simulink model "TB23_R2_SALS_Link"  (R2025a)
settings: Solver=FixedStepDiscrete  StartTime=0  StopTime=TB.t_end  FixedStep=TB.dt  RelTol=1e-3
InitFcn:
  | % 모델과 같은 폴더의 초기화 스크립트를 실행해 P(설계 파라미터)와 TB(시험 조건)를 만든다.
  | run(fullfile(fileparts(get_param(bdroot, 'FileName')), 'TB23_init.m'));
values from neighbouring files (symbols this model uses):
  TB = struct()    [TB23_init.m]    (also in run_TB23.m = evalin('base', 'TB'))
libraries: fl_lib x71, nesl_utility x31
(part 2 of 3)

== system TB23_R2_SALS_Link/StageB_Regulator/DAB_Primary/P3_leg2_high ==
  note: 스위치 셀: 이상 스위치(R_on, G_off) + 역병렬 바디 다이오드(Vf, R_d) + 출력용량 C_oss
      | 게이트: 전역 태그 "gD_P3" (> 0.5 이면 도통)
  C_oss : fl_lib/Electrical/Electrical Elements/Capacitor  c=Coss F  r=1e-6 Ohm  g=0 1/Ohm  i_specify=off  i_priority=None  i=0 A  i_nominal_specify=off  i_nominal_value=1  i_nominal_unit=A  v_specify=off  v_priority=None  v=0 V  v_nominal_specify=off  v_nominal_value=1  v_nominal_unit=V  vc_specify=off  vc_priority=High  vc=0 V  vc_nominal_specify=off  vc_nominal_value=1  vc_nominal_unit=V
  D_body : fl_lib/Electrical/Electrical Elements/Diode  Vf=Vf V  Ron=Rd Ohm  Goff=Goffd 1/Ohm  i_specify=off  i_priority=None  i=0 A  i_nominal_specify=off  i_nominal_value=1  i_nominal_unit=A  v_specify=off  v_priority=None  v=0 V  v_nominal_specify=off  v_nominal_value=1  v_nominal_unit=V
  Gate_PS : nesl_utility/Simulink-PS Converter  PhysicalDomain=network_engine_domain  SubClassName=ps_input  LeftPortType=input  RightPortType=output  PseudoPeriodic=off  Frequencies=[]  NoiseDistribution=none  NoiseParameters=[]  Unit=1  AffineConversion=off  FilteringAndDerivatives=zero  SimscapeFilterOrder=1  InputFilterTimeConstant=0.001  UdotUserProvided=0
  SW : fl_lib/Electrical/Electrical Elements/Switch  R_closed=Ron Ohm  G_open=Goff 1/Ohm  Threshold=0.5  i_specify=off  i_priority=None  i=0 A  i_nominal_specify=off  i_nominal_value=1  i_nominal_unit=A  v_specify=off  v_priority=None  v=0 V  v_nominal_specify=off  v_nominal_value=1  v_nominal_unit=V
  D : PMIOPort  Side=Left
  S : PMIOPort  Port=2  Side=Right
  wires:
  [gD_P3] -> Gate_PS/1
  connections:
  Gate_PS/RConn1 -- SW/RConn1
  SW/LConn1 -- D/RConn1 -- D_body/RConn1 -- C_oss/LConn1
  SW/RConn2 -- D_body/LConn1 -- S/RConn1 -- C_oss/RConn1

== system TB23_R2_SALS_Link/StageB_Regulator/DAB_Primary/P4_leg2_low ==
  note: 스위치 셀: 이상 스위치(R_on, G_off) + 역병렬 바디 다이오드(Vf, R_d) + 출력용량 C_oss
      | 게이트: 전역 태그 "gD_P4" (> 0.5 이면 도통)
  C_oss : fl_lib/Electrical/Electrical Elements/Capacitor  c=Coss F  r=1e-6 Ohm  g=0 1/Ohm  i_specify=off  i_priority=None  i=0 A  i_nominal_specify=off  i_nominal_value=1  i_nominal_unit=A  v_specify=off  v_priority=None  v=0 V  v_nominal_specify=off  v_nominal_value=1  v_nominal_unit=V  vc_specify=off  vc_priority=High  vc=0 V  vc_nominal_specify=off  vc_nominal_value=1  vc_nominal_unit=V
  D_body : fl_lib/Electrical/Electrical Elements/Diode  Vf=Vf V  Ron=Rd Ohm  Goff=Goffd 1/Ohm  i_specify=off  i_priority=None  i=0 A  i_nominal_specify=off  i_nominal_value=1  i_nominal_unit=A  v_specify=off  v_priority=None  v=0 V  v_nominal_specify=off  v_nominal_value=1  v_nominal_unit=V
  Gate_PS : nesl_utility/Simulink-PS Converter  PhysicalDomain=network_engine_domain  SubClassName=ps_input  LeftPortType=input  RightPortType=output  PseudoPeriodic=off  Frequencies=[]  NoiseDistribution=none  NoiseParameters=[]  Unit=1  AffineConversion=off  FilteringAndDerivatives=zero  SimscapeFilterOrder=1  InputFilterTimeConstant=0.001  UdotUserProvided=0
  SW : fl_lib/Electrical/Electrical Elements/Switch  R_closed=Ron Ohm  G_open=Goff 1/Ohm  Threshold=0.5  i_specify=off  i_priority=None  i=0 A  i_nominal_specify=off  i_nominal_value=1  i_nominal_unit=A  v_specify=off  v_priority=None  v=0 V  v_nominal_specify=off  v_nominal_value=1  v_nominal_unit=V
  D : PMIOPort  Side=Left
  S : PMIOPort  Port=2  Side=Right
  wires:
  [gD_P4] -> Gate_PS/1
  connections:
  Gate_PS/RConn1 -- SW/RConn1
  SW/LConn1 -- D/RConn1 -- D_body/RConn1 -- C_oss/LConn1
  SW/RConn2 -- D_body/LConn1 -- S/RConn1 -- C_oss/RConn1

== system TB23_R2_SALS_Link/StageB_Regulator/DAB_Secondary/S1_leg1_high ==
  note: 스위치 셀: 이상 스위치(R_on, G_off) + 역병렬 바디 다이오드(Vf, R_d) + 출력용량 C_oss
      | 게이트: 전역 태그 "gD_S1" (> 0.5 이면 도통)
  C_oss : fl_lib/Electrical/Electrical Elements/Capacitor  c=Coss F  r=1e-6 Ohm  g=0 1/Ohm  i_specify=off  i_priority=None  i=0 A  i_nominal_specify=off  i_nominal_value=1  i_nominal_unit=A  v_specify=off  v_priority=None  v=0 V  v_nominal_specify=off  v_nominal_value=1  v_nominal_unit=V  vc_specify=off  vc_priority=High  vc=0 V  vc_nominal_specify=off  vc_nominal_value=1  vc_nominal_unit=V
  D_body : fl_lib/Electrical/Electrical Elements/Diode  Vf=Vf V  Ron=Rd Ohm  Goff=Goffd 1/Ohm  i_specify=off  i_priority=None  i=0 A  i_nominal_specify=off  i_nominal_value=1  i_nominal_unit=A  v_specify=off  v_priority=None  v=0 V  v_nominal_specify=off  v_nominal_value=1  v_nominal_unit=V
  Gate_PS : nesl_utility/Simulink-PS Converter  PhysicalDomain=network_engine_domain  SubClassName=ps_input  LeftPortType=input  RightPortType=output  PseudoPeriodic=off  Frequencies=[]  NoiseDistribution=none  NoiseParameters=[]  Unit=1  AffineConversion=off  FilteringAndDerivatives=zero  SimscapeFilterOrder=1  InputFilterTimeConstant=0.001  UdotUserProvided=0
  SW : fl_lib/Electrical/Electrical Elements/Switch  R_closed=Ron Ohm  G_open=Goff 1/Ohm  Threshold=0.5  i_specify=off  i_priority=None  i=0 A  i_nominal_specify=off  i_nominal_value=1  i_nominal_unit=A  v_specify=off  v_priority=None  v=0 V  v_nominal_specify=off  v_nominal_value=1  v_nominal_unit=V
  D : PMIOPort  Side=Left
  S : PMIOPort  Port=2  Side=Right
  wires:
  [gD_S1] -> Gate_PS/1
  connections:
  Gate_PS/RConn1 -- SW/RConn1
  SW/LConn1 -- D/RConn1 -- D_body/RConn1 -- C_oss/LConn1
  SW/RConn2 -- D_body/LConn1 -- S/RConn1 -- C_oss/RConn1

== system TB23_R2_SALS_Link/StageB_Regulator/DAB_Secondary/S2_leg1_low ==
  note: 스위치 셀: 이상 스위치(R_on, G_off) + 역병렬 바디 다이오드(Vf, R_d) + 출력용량 C_oss
      | 게이트: 전역 태그 "gD_S2" (> 0.5 이면 도통)
  C_oss : fl_lib/Electrical/Electrical Elements/Capacitor  c=Coss F  r=1e-6 Ohm  g=0 1/Ohm  i_specify=off  i_priority=None  i=0 A  i_nominal_specify=off  i_nominal_value=1  i_nominal_unit=A  v_specify=off  v_priority=None  v=0 V  v_nominal_specify=off  v_nominal_value=1  v_nominal_unit=V  vc_specify=off  vc_priority=High  vc=0 V  vc_nominal_specify=off  vc_nominal_value=1  vc_nominal_unit=V
  D_body : fl_lib/Electrical/Electrical Elements/Diode  Vf=Vf V  Ron=Rd Ohm  Goff=Goffd 1/Ohm  i_specify=off  i_priority=None  i=0 A  i_nominal_specify=off  i_nominal_value=1  i_nominal_unit=A  v_specify=off  v_priority=None  v=0 V  v_nominal_specify=off  v_nominal_value=1  v_nominal_unit=V
  Gate_PS : nesl_utility/Simulink-PS Converter  PhysicalDomain=network_engine_domain  SubClassName=ps_input  LeftPortType=input  RightPortType=output  PseudoPeriodic=off  Frequencies=[]  NoiseDistribution=none  NoiseParameters=[]  Unit=1  AffineConversion=off  FilteringAndDerivatives=zero  SimscapeFilterOrder=1  InputFilterTimeConstant=0.001  UdotUserProvided=0
  SW : fl_lib/Electrical/Electrical Elements/Switch  R_closed=Ron Ohm  G_open=Goff 1/Ohm  Threshold=0.5  i_specify=off  i_priority=None  i=0 A  i_nominal_specify=off  i_nominal_value=1  i_nominal_unit=A  v_specify=off  v_priority=None  v=0 V  v_nominal_specify=off  v_nominal_value=1  v_nominal_unit=V
  D : PMIOPort  Side=Left
  S : PMIOPort  Port=2  Side=Right
  wires:
  [gD_S2] -> Gate_PS/1
  connections:
  Gate_PS/RConn1 -- SW/RConn1
  SW/LConn1 -- D/RConn1 -- D_body/RConn1 -- C_oss/LConn1
  SW/RConn2 -- D_body/LConn1 -- S/RConn1 -- C_oss/RConn1

== system TB23_R2_SALS_Link/StageB_Regulator/DAB_Secondary/S3_leg2_high ==
  note: 스위치 셀: 이상 스위치(R_on, G_off) + 역병렬 바디 다이오드(Vf, R_d) + 출력용량 C_oss
      | 게이트: 전역 태그 "gD_S3" (> 0.5 이면 도통)
  C_oss : fl_lib/Electrical/Electrical Elements/Capacitor  c=Coss F  r=1e-6 Ohm  g=0 1/Ohm  i_specify=off  i_priority=None  i=0 A  i_nominal_specify=off  i_nominal_value=1  i_nominal_unit=A  v_specify=off  v_priority=None  v=0 V  v_nominal_specify=off  v_nominal_value=1  v_nominal_unit=V  vc_specify=off  vc_priority=High  vc=0 V  vc_nominal_specify=off  vc_nominal_value=1  vc_nominal_unit=V
  D_body : fl_lib/Electrical/Electrical Elements/Diode  Vf=Vf V  Ron=Rd Ohm  Goff=Goffd 1/Ohm  i_specify=off  i_priority=None  i=0 A  i_nominal_specify=off  i_nominal_value=1  i_nominal_unit=A  v_specify=off  v_priority=None  v=0 V  v_nominal_specify=off  v_nominal_value=1  v_nominal_unit=V
  Gate_PS : nesl_utility/Simulink-PS Converter  PhysicalDomain=network_engine_domain  SubClassName=ps_input  LeftPortType=input  RightPortType=output  PseudoPeriodic=off  Frequencies=[]  NoiseDistribution=none  NoiseParameters=[]  Unit=1  AffineConversion=off  FilteringAndDerivatives=zero  SimscapeFilterOrder=1  InputFilterTimeConstant=0.001  UdotUserProvided=0
  SW : fl_lib/Electrical/Electrical Elements/Switch  R_closed=Ron Ohm  G_open=Goff 1/Ohm  Threshold=0.5  i_specify=off  i_priority=None  i=0 A  i_nominal_specify=off  i_nominal_value=1  i_nominal_unit=A  v_specify=off  v_priority=None  v=0 V  v_nominal_specify=off  v_nominal_value=1  v_nominal_unit=V
  D : PMIOPort  Side=Left
  S : PMIOPort  Port=2  Side=Right
  wires:
  [gD_S3] -> Gate_PS/1
  connections:
  Gate_PS/RConn1 -- SW/RConn1
  SW/LConn1 -- D/RConn1 -- D_body/RConn1 -- C_oss/LConn1
  SW/RConn2 -- D_body/LConn1 -- S/RConn1 -- C_oss/RConn1

== system TB23_R2_SALS_Link/StageB_Regulator/DAB_Secondary/S4_leg2_low ==
  note: 스위치 셀: 이상 스위치(R_on, G_off) + 역병렬 바디 다이오드(Vf, R_d) + 출력용량 C_oss
      | 게이트: 전역 태그 "gD_S4" (> 0.5 이면 도통)
  C_oss : fl_lib/Electrical/Electrical Elements/Capacitor  c=Coss F  r=1e-6 Ohm  g=0 1/Ohm  i_specify=off  i_priority=None  i=0 A  i_nominal_specify=off  i_nominal_value=1  i_nominal_unit=A  v_specify=off  v_priority=None  v=0 V  v_nominal_specify=off  v_nominal_value=1  v_nominal_unit=V  vc_specify=off  vc_priority=High  vc=0 V  vc_nominal_specify=off  vc_nominal_value=1  vc_nominal_unit=V
  D_body : fl_lib/Electrical/Electrical Elements/Diode  Vf=Vf V  Ron=Rd Ohm  Goff=Goffd 1/Ohm  i_specify=off  i_priority=None  i=0 A  i_nominal_specify=off  i_nominal_value=1  i_nominal_unit=A  v_specify=off  v_priority=None  v=0 V  v_nominal_specify=off  v_nominal_value=1  v_nominal_unit=V
  Gate_PS : nesl_utility/Simulink-PS Converter  PhysicalDomain=network_engine_domain  SubClassName=ps_input  LeftPortType=input  RightPortType=output  PseudoPeriodic=off  Frequencies=[]  NoiseDistribution=none  NoiseParameters=[]  Unit=1  AffineConversion=off  FilteringAndDerivatives=zero  SimscapeFilterOrder=1  InputFilterTimeConstant=0.001  UdotUserProvided=0
  SW : fl_lib/Electrical/Electrical Elements/Switch  R_closed=Ron Ohm  G_open=Goff 1/Ohm  Threshold=0.5  i_specify=off  i_priority=None  i=0 A  i_nominal_specify=off  i_nominal_value=1  i_nominal_unit=A  v_specify=off  v_priority=None  v=0 V  v_nominal_specify=off  v_nominal_value=1  v_nominal_unit=V
  D : PMIOPort  Side=Left
  S : PMIOPort  Port=2  Side=Right
  wires:
  [gD_S4] -> Gate_PS/1
  connections:
  Gate_PS/RConn1 -- SW/RConn1
  SW/LConn1 -- D/RConn1 -- D_body/RConn1 -- C_oss/LConn1
  SW/RConn2 -- D_body/LConn1 -- S/RConn1 -- C_oss/RConn1

== system TB23_R2_SALS_Link/StageB_Regulator/HBridge/QA_high ==
  note: 스위치 셀: 이상 스위치(R_on, G_off) + 역병렬 바디 다이오드(Vf, R_d) + 출력용량 C_oss
      | 게이트: 전역 태그 "gB_AH" (> 0.5 이면 도통)
  C_oss : fl_lib/Electrical/Electrical Elements/Capacitor  c=Coss F  r=1e-6 Ohm  g=0 1/Ohm  i_specify=off  i_priority=None  i=0 A  i_nominal_specify=off  i_nominal_value=1  i_nominal_unit=A  v_specify=off  v_priority=None  v=0 V  v_nominal_specify=off  v_nominal_value=1  v_nominal_unit=V  vc_specify=off  vc_priority=High  vc=0 V  vc_nominal_specify=off  vc_nominal_value=1  vc_nominal_unit=V
  D_body : fl_lib/Electrical/Electrical Elements/Diode  Vf=Vf V  Ron=Rd Ohm  Goff=Goffd 1/Ohm  i_specify=off  i_priority=None  i=0 A  i_nominal_specify=off  i_nominal_value=1  i_nominal_unit=A  v_specify=off  v_priority=None  v=0 V  v_nominal_specify=off  v_nominal_value=1  v_nominal_unit=V
  Gate_PS : nesl_utility/Simulink-PS Converter  PhysicalDomain=network_engine_domain  SubClassName=ps_input  LeftPortType=input  RightPortType=output  PseudoPeriodic=off  Frequencies=[]  NoiseDistribution=none  NoiseParameters=[]  Unit=1  AffineConversion=off  FilteringAndDerivatives=zero  SimscapeFilterOrder=1  InputFilterTimeConstant=0.001  UdotUserProvided=0
  SW : fl_lib/Electrical/Electrical Elements/Switch  R_closed=Ron Ohm  G_open=Goff 1/Ohm  Threshold=0.5  i_specify=off  i_priority=None  i=0 A  i_nominal_specify=off  i_nominal_value=1  i_nominal_unit=A  v_specify=off  v_priority=None  v=0 V  v_nominal_specify=off  v_nominal_value=1  v_nominal_unit=V
  D : PMIOPort  Side=Left
  S : PMIOPort  Port=2  Side=Right
  wires:
  [gB_AH] -> Gate_PS/1
  connections:
  Gate_PS/RConn1 -- SW/RConn1
  SW/LConn1 -- D/RConn1 -- D_body/RConn1 -- C_oss/LConn1
  SW/RConn2 -- D_body/LConn1 -- S/RConn1 -- C_oss/RConn1

== system TB23_R2_SALS_Link/StageB_Regulator/HBridge/QA_low ==
  note: 스위치 셀: 이상 스위치(R_on, G_off) + 역병렬 바디 다이오드(Vf, R_d) + 출력용량 C_oss
      | 게이트: 전역 태그 "gB_AL" (> 0.5 이면 도통)
  C_oss : fl_lib/Electrical/Electrical Elements/Capacitor  c=Coss F  r=1e-6 Ohm  g=0 1/Ohm  i_specify=off  i_priority=None  i=0 A  i_nominal_specify=off  i_nominal_value=1  i_nominal_unit=A  v_specify=off  v_priority=None  v=0 V  v_nominal_specify=off  v_nominal_value=1  v_nominal_unit=V  vc_specify=off  vc_priority=High  vc=0 V  vc_nominal_specify=off  vc_nominal_value=1  vc_nominal_unit=V
  D_body : fl_lib/Electrical/Electrical Elements/Diode  Vf=Vf V  Ron=Rd Ohm  Goff=Goffd 1/Ohm  i_specify=off  i_priority=None  i=0 A  i_nominal_specify=off  i_nominal_value=1  i_nominal_unit=A  v_specify=off  v_priority=None  v=0 V  v_nominal_specify=off  v_nominal_value=1  v_nominal_unit=V
  Gate_PS : nesl_utility/Simulink-PS Converter  PhysicalDomain=network_engine_domain  SubClassName=ps_input  LeftPortType=input  RightPortType=output  PseudoPeriodic=off  Frequencies=[]  NoiseDistribution=none  NoiseParameters=[]  Unit=1  AffineConversion=off  FilteringAndDerivatives=zero  SimscapeFilterOrder=1  InputFilterTimeConstant=0.001  UdotUserProvided=0
  SW : fl_lib/Electrical/Electrical Elements/Switch  R_closed=Ron Ohm  G_open=Goff 1/Ohm  Threshold=0.5  i_specify=off  i_priority=None  i=0 A  i_nominal_specify=off  i_nominal_value=1  i_nominal_unit=A  v_specify=off  v_priority=None  v=0 V  v_nominal_specify=off  v_nominal_value=1  v_nominal_unit=V
  D : PMIOPort  Side=Left
  S : PMIOPort  Port=2  Side=Right
  wires:
  [gB_AL] -> Gate_PS/1
  connections:
  Gate_PS/RConn1 -- SW/RConn1
  SW/LConn1 -- D/RConn1 -- D_body/RConn1 -- C_oss/LConn1
  SW/RConn2 -- D_body/LConn1 -- S/RConn1 -- C_oss/RConn1

== system TB23_R2_SALS_Link/StageB_Regulator/HBridge/QB_high ==
  note: 스위치 셀: 이상 스위치(R_on, G_off) + 역병렬 바디 다이오드(Vf, R_d) + 출력용량 C_oss
      | 게이트: 전역 태그 "gB_BH" (> 0.5 이면 도통)
  C_oss : fl_lib/Electrical/Electrical Elements/Capacitor  c=Coss F  r=1e-6 Ohm  g=0 1/Ohm  i_specify=off  i_priority=None  i=0 A  i_nominal_specify=off  i_nominal_value=1  i_nominal_unit=A  v_specify=off  v_priority=None  v=0 V  v_nominal_specify=off  v_nominal_value=1  v_nominal_unit=V  vc_specify=off  vc_priority=High  vc=0 V  vc_nominal_specify=off  vc_nominal_value=1  vc_nominal_unit=V
  D_body : fl_lib/Electrical/Electrical Elements/Diode  Vf=Vf V  Ron=Rd Ohm  Goff=Goffd 1/Ohm  i_specify=off  i_priority=None  i=0 A  i_nominal_specify=off  i_nominal_value=1  i_nominal_unit=A  v_specify=off  v_priority=None  v=0 V  v_nominal_specify=off  v_nominal_value=1  v_nominal_unit=V
  Gate_PS : nesl_utility/Simulink-PS Converter  PhysicalDomain=network_engine_domain  SubClassName=ps_input  LeftPortType=input  RightPortType=output  PseudoPeriodic=off  Frequencies=[]  NoiseDistribution=none  NoiseParameters=[]  Unit=1  AffineConversion=off  FilteringAndDerivatives=zero  SimscapeFilterOrder=1  InputFilterTimeConstant=0.001  UdotUserProvided=0
  SW : fl_lib/Electrical/Electrical Elements/Switch  R_closed=Ron Ohm  G_open=Goff 1/Ohm  Threshold=0.5  i_specify=off  i_priority=None  i=0 A  i_nominal_specify=off  i_nominal_value=1  i_nominal_unit=A  v_specify=off  v_priority=None  v=0 V  v_nominal_specify=off  v_nominal_value=1  v_nominal_unit=V
  D : PMIOPort  Side=Left
  S : PMIOPort  Port=2  Side=Right
  wires:
  [gB_BH] -> Gate_PS/1
  connections:
  Gate_PS/RConn1 -- SW/RConn1
  SW/LConn1 -- D/RConn1 -- D_body/RConn1 -- C_oss/LConn1
  SW/RConn2 -- D_body/LConn1 -- S/RConn1 -- C_oss/RConn1

== system TB23_R2_SALS_Link/StageB_Regulator/HBridge/QB_low ==
  note: 스위치 셀: 이상 스위치(R_on, G_off) + 역병렬 바디 다이오드(Vf, R_d) + 출력용량 C_oss
      | 게이트: 전역 태그 "gB_BL" (> 0.5 이면 도통)
  C_oss : fl_lib/Electrical/Electrical Elements/Capacitor  c=Coss F  r=1e-6 Ohm  g=0 1/Ohm  i_specify=off  i_priority=None  i=0 A  i_nominal_specify=off  i_nominal_value=1  i_nominal_unit=A  v_specify=off  v_priority=None  v=0 V  v_nominal_specify=off  v_nominal_value=1  v_nominal_unit=V  vc_specify=off  vc_priority=High  vc=0 V  vc_nominal_specify=off  vc_nominal_value=1  vc_nominal_unit=V
  D_body : fl_lib/Electrical/Electrical Elements/Diode  Vf=Vf V  Ron=Rd Ohm  Goff=Goffd 1/Ohm  i_specify=off  i_priority=None  i=0 A  i_nominal_specify=off  i_nominal_value=1  i_nominal_unit=A  v_specify=off  v_priority=None  v=0 V  v_nominal_specify=off  v_nominal_value=1  v_nominal_unit=V
  Gate_PS : nesl_utility/Simulink-PS Converter  PhysicalDomain=network_engine_domain  SubClassName=ps_input  LeftPortType=input  RightPortType=output  PseudoPeriodic=off  Frequencies=[]  NoiseDistribution=none  NoiseParameters=[]  Unit=1  AffineConversion=off  FilteringAndDerivatives=zero  SimscapeFilterOrder=1  InputFilterTimeConstant=0.001  UdotUserProvided=0
  SW : fl_lib/Electrical/Electrical Elements/Switch  R_closed=Ron Ohm  G_open=Goff 1/Ohm  Threshold=0.5  i_specify=off  i_priority=None  i=0 A  i_nominal_specify=off  i_nominal_value=1  i_nominal_unit=A  v_specify=off  v_priority=None  v=0 V  v_nominal_specify=off  v_nominal_value=1  v_nominal_unit=V
  D : PMIOPort  Side=Left
  S : PMIOPort  Port=2  Side=Right
  wires:
  [gB_BL] -> Gate_PS/1
  connections:
  Gate_PS/RConn1 -- SW/RConn1
  SW/LConn1 -- D/RConn1 -- D_body/RConn1 -- C_oss/LConn1
  SW/RConn2 -- D_body/LConn1 -- S/RConn1 -- C_oss/RConn1

== matlab function TB23_R2_SALS_Link/Load_CPL/SALS_Loads ==
  data: t input; i_load output; vb input; code input; prm input; p_load output
function [i_load, p_load] = prism_sals_loads(t, vb, code, prm)
%#codegen
%PRISM_SALS_LOADS  400 V 부하의 등급별 계약 응답(SALS 메시지 지연·손실·워치독 포함). TB23부터.
%
%   검증 코드 sals_loads.SalsLoads(E29)와 같은 해석식이다. 보호 상태기계(ctrl/prism_r2_supervisor.m, SALS 모드)가
%   s(10)에 비트로 명령을 낸다: 1 접촉기 열림(400 V급 부하 분리), 2 SALS 감발, 4 SALS 되돌림, 8 Stage C 회생 차단,
%   16 Stage A 정지(이 블록은 쓰지 않음). 비트가 처음 켜진 시각을 명령 시각으로 잡는다.
%     M0  Stage C sc(회생 차단이면 t_sc 뒤 하한 0으로 sc_slew 변화율), V2L v2l(계단, SALS로 줄이지 않음)
%     M1  컴프레서 comp, D  PTC ptc·배터리 히터 bh:
%         감발 도착 = 명령 + 재송신 주기 × (앞의 손실 수) + 지연. 손실 수 −1이면 모두 손실(도착 없음).
%         D는 워치독으로 명령 + wd에 0으로 간다(마지막 유효 수신 ≤ 명령 시각). 도착 뒤 감소 변화율 dn으로 0까지.
%         되돌림 도착 뒤 증가 변화율 up으로 요청값까지(되돌림이 감발보다 먼저 도착하면 감발은 버려진다).
%     접촉기 열림이면 Stage C만 남는다. 버스가 v_cut 아래면 모든 부하가 끊긴다(검증 코드 E17의 저전압 차단).
%
%   입력  t 시각 [s], vb 버스전압(한 간격 지연·시작 보호), code s(10) 비트 명령,
%         prm [sc v2l comp ptc bh | d_comp d_ptc d_bh | k_comp k_ptc k_bh | kr_comp kr_ptc kr_bh |
%              period wd up dn t_sc sc_slew v_min v_cut]  (22개, 시간 [s]·변화율 [W/s]는 시간 축소를 이미 넣은 값)
%   출력  i_load = p_load / max(vb, v_min) [A], p_load [W]

persistent t_cut t_rest t_blk acut arest
if isempty(t_cut)
    t_cut = -1; t_rest = -1; t_blk = -1; acut = inf(3, 1); arest = inf(3, 1);
end
mix = prm(1:5); dl = prm(6:8); kc = prm(9:11); kr = prm(12:14);
period = prm(15); wd = prm(16); up = prm(17); dn = prm(18); t_sc = prm(19); sc_slew = prm(20); vmin = prm(21); vcut = prm(22);
c = round(code);
open_c = mod(c, 2) >= 1; cut = mod(floor(c/2), 2) >= 1; rest = mod(floor(c/4), 2) >= 1; blk = mod(floor(c/8), 2) >= 1;

if cut && t_cut < 0                                   % 감발 명령: 장치별 도착 시각
    t_cut = t;
    for j = 1:3
        if kc(j) < 0, a = inf; else, a = t + kc(j)*period + dl(j); end
        if j >= 2, a = min(a, t + wd); end            % D(PTC·배터리 히터) 워치독
        acut(j) = a;
    end
end
if (blk || cut) && t_blk < 0
    t_blk = t;
end
if rest && t_rest < 0 && t_cut >= 0                   % 되돌림 명령
    t_rest = t;
    for j = 1:3
        if kr(j) < 0, arest(j) = inf; else, arest(j) = t + kr(j)*period + dl(j); end
    end
end

% Stage C(M0): 회생 차단이면 하한 0으로
sc = mix(1);
if sc < 0 && t_blk >= 0 && t >= t_blk + t_sc
    sc = min(0, sc + sc_slew*(t - t_blk - t_sc));
end
p = sc;
if ~open_c
    p = p + mix(2);
    for j = 1:3
        p0 = mix(2 + j); ac = acut(j); ar = arest(j);
        if t < ac || ar <= ac
            pj = p0;
        else
            pj = max(p0 - dn*(t - ac), 0);
            if t >= ar
                pa = max(p0 - dn*(ar - ac), 0);
                pj = min(p0, pa + up*(t - ar));
            end
        end
        p = p + pj;
    end
end
if vb < vcut
    p = 0;
end
p_load = p;
i_load = p/max(vb, vmin);
end

== matlab function TB23_R2_SALS_Link/StageA_Stop ==
  data: code input; R output; prm input
function R = prism_stageA_stop(code, prm)
%#codegen
%PRISM_STAGEA_STOP  Stage A 협조 정지 스위치(TB23): 보호 상태기계 비트 명령 16(Stage A 정지)이면 V_A 등가 전원을 끊는다.
%
%   Stage A는 이상 전원 V_bat/2로 등가했다. 정지하면 모든 위상이 자연 턴오프로 꺼지고 V_A 노드는 출력 커패시터 C_A만 남는다
%   (검증 코드 E17 r2_run의 astop: V_A = C_A가 경로전류로 방전). 이 블록은 전원과 C_A 노드 사이 가변 저항 값을 낸다.
%   입력  code  상태기계 s(10)(SALS 모드 비트 명령), prm [R_on R_off] [Ω]
%   출력  R     R_on(동작) 또는 R_off(정지)
c = round(code);
if mod(floor(c/16), 2) >= 1
    R = prm(2);
else
    R = prm(1);
end
end

== matlab function TB23_R2_SALS_Link/DAB_Loss_Model/DAB_Loss ==
  data: t input; iloss output; vl input; il input; iL input; vb input; prm input; ploss0 input
function iloss = prism_dab_loss(t, vl, il, iL, vb, prm, ploss0)
%#codegen
%PRISM_DAB_LOSS  DAB 손실 등가 전류(검증 모델과 같은 손실 모델).
%
%   스위칭 회로의 DAB에는 권선저항 R_dab만 있고 스위칭·자기 손실이 없다. 검증 모델(E12)은 평균모델과 같은
%   방향별 효율 η = 0.96을 쓰기 위해, 직전 제어주기의 평균 링크전력 p̄로 정한 손실
%       P_loss = (1/η − 1)·max(p̄, 0) + (1 − η)·max(−p̄, 0) − R_dab·mean(i_L²)   (0 이상)
%   을 버스에서 끄는 전류 P_loss/v_bus로 넣는다. 이 블록은 같은 계산을 해서 버스의 제어 전류원에 준다.
%   이렇게 하면 정상상태의 DAB 총손실이 검증 모델과 같아, 두 모델의 차이는 스위칭 동작에서만 나온다.
%
%   입력  t 시각, vl 링크전압, il 링크 직류전류(2차 브리지 → 링크), iL 누설 전류, vb 버스전압
%         prm [dt Np η R_dab]   ploss0 초기 손실 [W](평형점 링크전력 기준)
%   출력  iloss  버스에서 끄는 손실 전류 [A]

persistent accP accI2 ploss started
if isempty(started)
    started = 1; accP = 0; accI2 = 0; ploss = ploss0;
end
dt = prm(1); Np = round(prm(2)); eta = prm(3); Rd = prm(4);
k = round(t/dt);
accP = accP + vl*il;
accI2 = accI2 + iL*iL;
if mod(k, Np) == Np - 1                       % 주기 마지막 간격에서 갱신(다음 주기에 적용)
    pbar = accP/Np;
    lossEta = (1/eta - 1)*max(pbar, 0) + (1 - eta)*max(-pbar, 0);
    ploss = max(lossEta - Rd*accI2/Np, 0);
    accP = 0; accI2 = 0;
end
iloss = ploss/max(vb, 1);
end

== matlab function TB23_R2_SALS_Link/Controller_StageB/R2_Supervisor ==
  data: t input; s output; y input; fl input; prm input; smp input
function s = prism_r2_sup_sampler(t, y, fl, prm, smp)
%#codegen
%PRISM_R2_SUP_SAMPLER  R2 보호 상태기계 표본화 실행기(TB09, MATLAB Function 블록의 진입 함수).
%
%   5 µs마다(제어기와 같은 표본 시점, 제어기보다 먼저) ctrl/prism_r2_supervisor.m을 한 번 계산하고 그 밖에는 직전 출력을 유지한다.
%   입력  t 시각, y [i_p v_s v_bus i_h v_link], fl [게이트 구동기 고장 신호, 비교기 차단 래치](한 간격 지연),
%         prm 상태기계 파라미터(TB.sup_prm), smp [dt Np]
%   출력  s 상태기계 지령 12개(prism_r2_supervisor.m 참조)

persistent sh
if isempty(sh)
    sh = zeros(12, 1);
end
k = round(t/smp(1));
if mod(k, round(smp(2))) == 0
    sh = prism_r2_supervisor(t, y, fl, prm);
end
s = sh;
end

function s = prism_r2_supervisor(t, y, fl, prm)
%#codegen
%PRISM_R2_SUPERVISOR  R2 창 조정 모듈의 측정 기반 보호 상태기계(TB09, 검증 코드 E17 r2_run의 상태기계와 같은 논리).
%
%  5 µs마다(호출 측 표본기) 측정값과 고장 신호로 운전 상태를 정하고, 제어기·게이트·바이패스·제동 저항·부하 분리 명령을 낸다.
%  상태 번호
%    0 바이패스          바이패스 닫힘, H-브리지·DAB 정지(버스 = V_A)
%    1 준비(PREP)        바이패스 + H-브리지(영벡터 또는 전류 조향: 바이패스 전류 → 0)
%    2 열림 대기         바이패스 열림, H-브리지 영벡터(또는 조향) → t_wait 뒤 제어 시작
%    3 창 조정           채택 제어기(기준 V_A → V_W 램프 뒤 V_W)
%    4 끔 램프 / 5 끔 유지(기준 = V_A 추정, |v_s| ≤ 2 V가 50 µs 이어지면) / 6 영벡터(또는 직렬전압 조향) → 바이패스
%    7 DAB 고장 유지     H-브리지는 계속 조정, DAB 정지, 링크 제동 저항으로 링크 ≤ 110 V, 400 V 부하 분리 대기
%    8 DAB 고장 램프     기준 → V_A(1 ms) → V_A 추정 추종, |v_s| ≤ 2 V가 50 µs 이어지면 → 6 → 강등
%    9 H-브리지 고장 유지  H-브리지 꺼짐(다이오드 정류), DAB 보조 루프가 링크전압으로 버스를 V_W에 붙잡음 + 제동 저항
%   10 링크 붕괴         링크 기준을 20 V/ms로 0 V까지 → 직렬전압이 다이오드 전압까지 줄어듦.
%                        링크 ≤ VL_SOFT, 또는 정체(기준 0 도달 뒤 T_STALL 동안 DV_STALL도 안 내려가고 링크 ≤ VL_STALL), 또는 T_COL_MAX → 11
%   11 소프트 바이패스   바이패스 저항을 10 Ω에서 로그 램프로 낮추되(제한 없으면 T_SOFT에 3.3 mΩ), 경로전류가 투입 시작값 + DI_SOFT를
%                        넘으면 표본마다 K_UP배로 되올린다(경로전류 조절). 3.3 mΩ에 이르거나 T_SOFT_MAX가 지나면 → 12
%   12 강등              바이패스 닫힘, Stage B 정지(버스 = V_A)
%   13 이중 고장         DAB 고장 중 H-브리지 차단: Stage A 협조 정지가 필요(이 모델 밖)
%
%  (2026-10-24 TB09 1차 결과로 추가: 회로에서는 링크 붕괴가 3.5–22 V에서 멈췄고, 남은 직렬전압을 로그 램프로 닫자 경로전류가
%   177 A까지 올랐다. 그래서 정체 감지와 경로전류 조절을 넣었다. 같은 논리를 검증 코드 E17에도 넣었다.)
%
%  (2026-10-24 TB10, 검증 코드 E20: prm이 60개면 다음을 켠다. 56개(TB09)면 이전과 같다.)
%   prm(57) 전압비 정합 유지(1): H-브리지 강등 유지(9)의 링크 기준 = (V_A − (R + R_h)i_p − 2V_D)/(n + 1), 제동 저항은 기준 추종
%   prm(58) 일시 감발(1): H-브리지 고장이면 V_A와 무관하게 400 V 부하 출력을 줄이고, V_A ≤ 상한이면 강등 T_RESTORE 뒤 되돌림
%   prm(59) 소프트 투입 시간 상한이면 주 스위치를 닫지 않고 이중 고장(13)으로
%   prm(60) T_RESTORE [s]
%   DAB 변조(EPS)와 첨두 상한은 게이트 쪽 ctrl/prism_dab_eps_map.m이 맡는다(상태 9–11, DAB 모드 1).
%
%  (2026-10-28 TB23, 검증 코드 E29: prm이 69개면 SALS 연동 모드. 60개 이하면 이전과 같다.)
%   prm(61) SALS 모드(1): 고장 검출 때 SALS 감발 + Stage C 회생 차단을 내고, V_A > 상한 − 2 V면 접촉기 분리도 바로 명령한다.
%           감발 전용(V_A ≤ 상한 − 2 V)이면 유지(9)를 부하전류 추정 i_load = i_p − C_tot·dv_bus/dt(τ_il 필터)가 |i_load| ≤ I_COL로
%           T_CONF 이어질 때 끝내고, T_CUR_MAX 안에 안 되면 접촉기 분리로 넘어간다. 강등 T_RESTORE 뒤 SALS 되돌림(접촉기를 연 경우는 없음).
%           (고장 직후 다이오드가 막힌 동안은 버스 커패시터가 부하를 대므로 경로전류만으로는 판단할 수 없다.)
%           이중 고장(13)이면 접촉기 분리 + SALS 감발, ASTOP 뒤 Stage A 정지, (FS_BRAKE) 링크 제동 저항 과전압 보호 유지.
%   prm(62) I_COL [A], prm(63) T_CONF [s], prm(64) T_CUR_MAX [s], prm(65) FS_BRAKE(1), prm(66) ASTOP [s](< 0이면 Stage A 정지 없음),
%   prm(67) C_tot = C_b + C_dmp [F], prm(68) τ_il [s], prm(69) 부하전류 추정 시작값 [A]
%   SALS 모드의 s(10)은 비트 명령이다: 1 접촉기 열림(분리 끝), 2 SALS 감발, 4 SALS 되돌림, 8 Stage C 회생 차단, 16 Stage A 정지
%   (부하 블록 ctrl/prism_sals_loads.m, Stage A 정지 스위치가 읽는다).
%
%  입력  t    시각 [s]
%        y    측정 [i_p v_s v_bus i_h v_link]
%        fl   [게이트 구동기 고장 신호(H-브리지 개방), 하드웨어 비교기 차단 래치]
%        prm  파라미터 벡터(TB09_init.m의 TB.sup_prm, 번호는 아래 코드 주석)
%  출력  s = [V_ref; 재초기화; 브리지 모드(0 제어 PWM, 1 영벡터, 2 차단, 3 조향 PWM); 조향 변조율;
%             DAB 모드(0 제어기, 1 보조 지령, 2 정지); 보조 링크전류 지령; 바이패스 소프트 저항 [Ω]; 바이패스 주 스위치(1/0);
%             제동 저항 게이트(1/0); 400 V 부하 분리(1/0); 상태 번호; 고장 검출(0 없음, 1 구동기, 2 비교기, 3 링크 창, 4 버스 창)]

persistent st t_st t_det det shed_cmd shed sw_since vb_since rv0 rv1 rt1 rtype qb amode vl0 t0 tsoft0 Rs main brk mst gsince ip_s0 stall_t stall_v ...
           curt_only restored t_cont low_since cutb restb blkb t_as il_f vb_prev
VW = prm(1); upper = prm(2); H = prm(3); R = prm(4); Rh = prm(5); Cs = prm(6); Lh = prm(7); itau = prm(8);
Clink = prm(9); VD = prm(10); t_ev = prm(11); ev = prm(12); pol = prm(13); prep = prm(14); cls = prm(15);
t_prep = prm(16); t_wait = prm(17); RAMP = prm(18); HOLD = prm(19); ZERO = prm(20); t_shed = prm(21);
RATE = prm(22); VL_SOFT = prm(23); T_SOFT = prm(24); R_SOFT0 = prm(25); R_ON = prm(26); T_COL_MAX = prm(27);
VL_LO = prm(28); VL_HI = prm(29); T_SW = prm(30); VB_SW = prm(31); T_VB = prm(32);
KP_B = prm(33); KI_B = prm(34); QB_MAX = prm(35); W_L = prm(36); TAU_ST = prm(37); R_OPEN = prm(38);
P_r = prm(39); link_max = prm(40); turns = prm(41); phmax = prm(42); fs = prm(43); Ldab = prm(44); vbat = prm(45);
st0 = prm(46); Ts = prm(47); VS_GATE = prm(48); T_GATE = prm(49); T_GATE_MAX = prm(50);
VL_STALL = prm(51); T_STALL = prm(52); DV_STALL = prm(53); DI_SOFT = prm(54); K_UP = prm(55); T_SOFT_MAX = prm(56);
K_DN = (R_SOFT0/R_ON)^(Ts/T_SOFT);                    % 제한에 안 걸리면 10 Ω → 3.3 mΩ를 T_SOFT에 지나는 표본당 비율
HOLD_MATCH = 0; CURTAIL = 0; SOFT_FAIL = 0; T_RESTORE = 0.5e-3;
if numel(prm) >= 60
    HOLD_MATCH = prm(57); CURTAIL = prm(58); SOFT_FAIL = prm(59); T_RESTORE = prm(60);
end
SALS = 0; I_COL = 0; T_CONF = 0; T_CUR_MAX = 0; FS_BRAKE = 0; ASTOP = -1; C_TOT = 0; TAU_IL = 1; IL0 = 0;
if numel(prm) >= 69
    SALS = prm(61); I_COL = prm(62); T_CONF = prm(63); T_CUR_MAX = prm(64); FS_BRAKE = prm(65); ASTOP = prm(66);
    C_TOT = prm(67); TAU_IL = prm(68); IL0 = prm(69);
end

ip = y(1); vs = y(2); vb = y(3); ih = y(4); vl = y(5);
if isempty(st)
    st = st0; t_st = 0; t_det = -1; det = 0; shed_cmd = -1; shed = 0; sw_since = -1; vb_since = -1;
    rv0 = VW; rv1 = VW; rt1 = 0; rtype = 0; qb = 0; amode = 0; vl0 = 100; t0 = 0; tsoft0 = 0;
    if st0 == 3, Rs = R_OPEN; main = 0; else, Rs = R_OPEN; main = 1; end
    brk = 0; mst = 0; gsince = -1; ip_s0 = 0; stall_t = -1; stall_v = 0; curt_only = 0; restored = 0;
    t_cont = -1; low_since = -1; cutb = 0; restb = 0; blkb = 0; t_as = -1; il_f = IL0; vb_prev = vb;
end
va_m = vbat/2 - R*ip;                                  % V_A 추정(배터리 전압 센서 − 경로 강하)
gwin = (st == 5 && t - t_st >= HOLD - 1e-12) || (st == 8 && t - t_st >= RAMP + HOLD - 1e-12);
if gwin && abs(vs) <= VS_GATE                          % 영벡터 진입 조건: 최소 유지 뒤 |v_s| ≤ 2 V가 50 µs 이어짐
    if gsince < 0, gsince = t; end
else
    gsince = -1;
end
gate_ok = gsince >= 0 && t - gsince >= T_GATE - 1e-12;
bridge_dead = fl(1) > 0.5 || fl(2) > 0.5;
% ---- 고장 검출 --------------------------------------------------------------------------------
if t_det < 0
    if fl(1) > 0.5, t_det = t; det = 1; end
    if fl(2) > 0.5, t_det = t; det = 2; end
    if t_det < 0 && (st == 3 || st == 4 || st == 5)
        if vl < VL_LO || vl > VL_HI
            if sw_since < 0, sw_since = t; end
            if t - sw_since >= T_SW - 1e-12, t_det = t; det = 3; end
        else
            sw_since = -1;
        end
        if abs(vb - vref_at(t, rtype, rv0, rv1, rt1, RAMP, VW, va_m)) > VB_SW
            if vb_since < 0, vb_since = t; end
            if t - vb_since >= T_VB - 1e-12, t_det = t; det = 4; end
        else
            vb_since = -1;
        end
    end
elseif fl(2) > 0.5 && det == 3 && st ~= 13 && st ~= 12 && st >= 6 && st <= 8
    st = 13; t_st = t;                                  % DAB 고장 강등 중 하드웨어 차단 → 이중 고장
end
sw_states = (st >= 1 && st <= 8);
hb_det = det == 1 || det == 2 || det == 4;
if t_det >= 0 && shed_cmd < 0 && st ~= 0 && (va_m > upper - 2 || (CURTAIL > 0.5 && hb_det))
    shed_cmd = t;
    curt_only = double(va_m <= upper - 2);              % 상한 안이면 일시 감발(강등 뒤 되돌림)
    if SALS > 0.5                                       % (E29) SALS 감발은 항상, 접촉기 분리는 상한을 넘는 팩만 바로
        cutb = 1;
        if curt_only < 0.5, t_cont = t; end
    end
end
if SALS > 0.5
    if t_det >= 0, blkb = 1; end                        % Stage C 회생 차단(허브 내부 명령)
    if st == 13 && t_cont < 0
        cutb = 1; t_cont = t;                           % 이중 고장: 접촉기 분리 + SALS 감발
    end
    if st == 13 && ASTOP >= 0 && t_as < 0
        t_as = t + ASTOP;                               % 이중 고장: Stage A 정지
    end
end
if SALS > 0.5                                           % (E29) 부하전류 추정(경로전류 − 버스 커패시터 전류)
    il_f = il_f + ((ip - C_TOT*(vb - vb_prev)/Ts) - il_f)*Ts/TAU_IL; vb_prev = vb;
end
cur_ok = false;                                         % (E29) 감발 전용: 부하전류 추정으로 유지(9) 끝, 시간 상한이면 접촉기 분리
if SALS > 0.5 && st == 9 && curt_only > 0.5 && t_cont < 0
    if abs(il_f) <= I_COL
        if low_since < 0, low_since = t; end
        cur_ok = t - low_since >= T_CONF - 1e-12;
    else
        low_since = -1;
    end
    if ~cur_ok && t - shed_cmd >= T_CUR_MAX - 1e-12
        t_cont = t;
    end
end
if SALS > 0.5
    if t_cont >= 0 && t - t_cont >= t_shed - 1e-12
        shed = 1;                                       % 접촉기 열림(분리 끝)
    end
    if curt_only > 0.5 && t_cont < 0 && st == 12 && restored < 0.5 && t - t_st >= T_RESTORE - 1e-12
        restored = 1; restb = 1;                        % SALS 되돌림
    end
else
    if shed_cmd >= 0 && t - shed_cmd >= t_shed - 1e-12 && restored < 0.5
        shed = 1;
    end
    if curt_only > 0.5 && st == 12 && restored < 0.5 && t - t_st >= T_RESTORE - 1e-12
        shed = 0; restored = 1;                         % 버스 = V_A ≤ 상한: 400 V 부하 출력 되돌림
    end
end
% ---- 강등 경로 선택 ----------------------------------------------------------------------------
if (det == 1 || det == 2 || det == 4) && sw_states && st ~= 13
    if pol == 1                                          % 즉시 바이패스(비교용)
        main = 1; Rs = R_OPEN; st = 12; t_st = t;
    elseif pol == 2                                      % 바로 붕괴(비교용)
        amode = 1; t0 = t; vl0 = vl; st = 10; t_st = t;
    else
        st = 9; t_st = t; amode = 0; qb = 0;
    end
elseif det == 3 && (st == 3 || st == 4 || st == 5)
    if pol == 2 && shed_cmd >= 0                         % 제동 저항으로 유지
        st = 7; t_st = t;
    else
        rv0 = vref_at(t, rtype, rv0, rv1, rt1, RAMP, VW, va_m); rv1 = va_m; rt1 = t; rtype = 1; st = 8; t_st = t;
    end
end
% ---- 링크 붕괴 정체 감지(기준이 0에 닿은 뒤) ------------------------------------------------------------
stalled = false;
if st == 10 && t - t_st >= vl0/RATE - 1e-12
    if stall_t < 0 || stall_v - vl >= DV_STALL
        stall_t = t; stall_v = vl;
    end
    stalled = (t - stall_t >= T_STALL - 1e-12) && vl <= VL_STALL;
end
% ---- 정상 순서와 강등 진행 --------------------------------------------------------------------------
if st == 0 && ev == 1 && t >= t_ev && vbat/2 >= VW + H
    st = 1; t_st = t;
elseif st == 1 && t - t_st >= t_prep - 1e-12
    main = 0; Rs = R_OPEN; st = 2; t_st = t;
elseif st == 2 && t - t_st >= t_wait - 1e-12
    rv0 = va_m; rv1 = VW; rt1 = t; rtype = 1; st = 3; t_st = t;
elseif st == 3 && ev == 2 && t >= t_ev && t_det < 0 && vbat/2 <= VW - H
    rv0 = vref_at(t, rtype, rv0, rv1, rt1, RAMP, VW, va_m); rv1 = va_m; rt1 = t; rtype = 1; st = 4; t_st = t;
elseif st == 4 && t - t_st >= RAMP - 1e-12
    rtype = 2; st = 5; t_st = t;                         % 램프 뒤에는 기준이 V_A 추정을 따라간다
elseif st == 5 && t - t_st >= HOLD - 1e-12 && (gate_ok || t - t_st >= T_GATE_MAX - 1e-12)
    st = 6; t_st = t;
elseif st == 7 && shed > 0.5
    rv0 = vref_at(t, rtype, rv0, rv1, rt1, RAMP, VW, va_m); rv1 = va_m; rt1 = t; rtype = 1; st = 8; t_st = t;
elseif st == 8 && t - t_st >= RAMP - 1e-12 && rtype ~= 2
    rtype = 2;
elseif st == 8 && t - t_st >= RAMP + HOLD - 1e-12 && (gate_ok || t - t_st >= RAMP + T_GATE_MAX - 1e-12)
    st = 6; t_st = t;
elseif st == 6 && t - t_st >= ZERO - 1e-12
    main = 1; Rs = R_OPEN;
    if t_det >= 0, st = 12; else, st = 0; end
    t_st = t;
elseif st == 9 && (shed_cmd < 0 || shed > 0.5 || cur_ok)
    amode = 1; t0 = t; vl0 = vl; st = 10; t_st = t;
elseif st == 10 && (vl <= VL_SOFT || stalled || t - t_st >= T_COL_MAX - 1e-12)
    if pol == 5
        main = 1; Rs = R_OPEN; st = 12;
    else
        tsoft0 = t; ip_s0 = ip; Rs = R_SOFT0; st = 11;
    end
    t_st = t;
elseif st == 11 && (Rs <= R_ON*(1 + 1e-9) || t - t_st >= T_SOFT_MAX - 1e-12)
    if Rs > R_ON*(1 + 1e-9) && SOFT_FAIL > 0.5
        st = 13; t_st = t;                              % 시간 상한: 닫지 않고 이중 고장(Stage A 협조 정지)
    else
        main = 1; Rs = R_OPEN; st = 12; t_st = t;
    end
end
if st == 11 && t > tsoft0 + 1e-12                        % 소프트 투입(경로전류 조절)
    if ip > ip_s0 + DI_SOFT
        Rs = min(Rs*K_UP, R_SOFT0);
    else
        Rs = max(Rs/K_DN, R_ON);
    end
end
% ---- 지령 --------------------------------------------------------------------------------------
vref = vref_at(t, rtype, rv0, rv1, rt1, RAMP, VW, va_m);
rst = double(st == 0 || st == 1 || st == 2 || st == 6 || st >= 9);
steer = (st == 1 || st == 2) && prep > 0.5 || (st == 6 && cls > 0.5);
if st == 3 || st == 4 || st == 5 || st == 7 || st == 8
    bmode = 0;
elseif steer
    bmode = 3;
elseif st == 1 || st == 2 || st == 6
    bmode = 1;
else
    bmode = 2;
end
if bridge_dead, bmode = 2; end
if steer
    if st == 6, ihs = ip - Cs*vs/TAU_ST; else, ihs = ip; end
    mst = min(max((vs + Rh*ih + Lh/itau*(ihs - ih))/max(vl, 1), -0.95), 0.95);
end
% 보조 링크 루프(H-브리지 강등 9–11)
icmd_aux = 0; vlr = vl;
if st >= 9 && st <= 11
    if amode == 0 && HOLD_MATCH > 0.5
        vlr = min(max((vbat/2 - (R + Rh)*ip - 2*VD)/(turns + 1), 0), 100);   % DAB 전압비 정합(n·v_link = v_bus)
    elseif amode == 0
        e = vb - VW;
        qb = min(max(qb + Ts*KI_B*e, -QB_MAX), QB_MAX);
        ff = vbat/2 - (R + Rh)*ip - 2*VD - VW;
        vlr = min(max(ff + KP_B*e + qb, 0), 110);
    else
        vlr = max(vl0 - RATE*(t - t0), 0);
    end
    sps = max(vb, 0)*turns*phmax*(1 - phmax/pi)/(2*pi*fs*Ldab);
    lim = min([link_max, sps, P_r/max(vl, 1e-3)]);
    icmd_aux = min(max(-abs(ih) + Clink*W_L*(vlr - vl), -lim), lim);
end
if st >= 9 && st <= 11
    dmode = 1;
elseif st == 3 || st == 4 || st == 5 || st == 7 || st == 8
    dmode = 0;
else
    dmode = 2;
end
if det == 3, dmode = 2; end                              % DAB 고장: DAB 게이트는 고장 주입으로 이미 꺼져 있음
% 제동 저항(정책 4·5, DAB 정책 2). H-브리지 강등 유지(9) 중에는 링크 과전압 보호만(110 V), 붕괴·소프트 투입(10·11) 중에는
% 링크 기준 + 5 V 위에서 켠다(2026-10-24: 유지 중 기준 추종 제동은 경로전류 첨두를 키워 E17에서 W410 103 A로 불통과)
if (pol == 4 || pol == 5) && st == 9 && HOLD_MATCH < 0.5
    if vl > 110, brk = 1; elseif vl < 105, brk = 0; end
elseif (pol == 4 || pol == 5) && st == 9
    if vl > vlr + 5, brk = 1; elseif vl < vlr + 2, brk = 0; end   % 정합 유지: DAB 정격 밖 전력을 제동 저항이
elseif (pol == 4 || pol == 5) && st >= 10 && st <= 11
    if vl > vlr + 5, brk = 1; elseif vl < vlr + 2, brk = 0; end
elseif pol == 2 && det == 3 && (st == 7 || st == 8 || st == 6)
    if vl > 110, brk = 1; elseif vl < 105, brk = 0; end
elseif st == 13 && FS_BRAKE > 0.5                        % (E29) 이중 고장에서도 링크 과전압 보호
    if vl > 110, brk = 1; elseif vl < 105, brk = 0; end
else
    brk = 0;
end
shed_out = shed;
if SALS > 0.5                                            % 비트 명령(부하 블록·Stage A 정지 스위치)
    shed_out = shed + 2*cutb + 4*restb + 8*blkb + 16*double(t_as >= 0 && t >= t_as - 1e-12);
end
s = [vref; rst; bmode; mst; dmode; icmd_aux; Rs; main; brk; shed_out; st; det];
end

function v = vref_at(t, rtype, v0, v1, t1, RAMP, VW, va_m)
% 기준전압: 0 = V_W, 1 = v0 → v1 직선 램프(RAMP), 2 = V_A 추정 추종(끔·DAB 고장 램프 뒤)
if rtype < 0.5
    v = VW;
elseif rtype < 1.5
    v = v0 + (v1 - v0)*min((t - t1)/RAMP, 1);
else
    v = va_m;
end
end

== matlab function TB23_R2_SALS_Link/Controller_StageB/Adopted_Controller ==
  data: t input; u output; y input; prm input; init input; tab input; smp input; dg output
function [u, dg] = prism_ctrl_sampler_r2b(t, y, prm, init, tab, smp)
%#codegen
%PRISM_CTRL_SAMPLER_R2B  채택 제어기 표본화 실행기의 R2 보호 상태기계판(TB09, MATLAB Function 블록의 진입 함수).
%
%   ctrl/prism_ctrl_sampler_r2.m과 같이 5 µs마다 제어기를 한 번 계산하고, 상태기계(ctrl/prism_r2_supervisor.m)의
%   지령을 함께 받는다.
%     y(10) V_ref, y(11) 재초기화, y(12) 브리지 모드(3이면 상태기계의 조향 변조율을 PWM 비교값으로),
%     y(13) 조향 변조율, y(14) DAB 모드(1이면 보조 링크전류 지령), y(15) 보조 링크전류 지령
%   제어 법칙은 prism_stageB_controller.m 그대로다(보조 지령은 링크전압 PI 대신 들어간다).
%
%   입력  y = [i_p v_s v_bus i_h v_link V_bat i_link_avg φ_c0 φ_c1 | 상태기계 지령 6개]
%   출력  u, dg : ctrl/prism_ctrl_sampler.m과 같음

persistent uh dgh
if isempty(uh)
    uh = [init(3); 0];
    dgh = zeros(6, 1);
end
k = round(t/smp(1));
if mod(k, round(smp(2))) == 0
    prm2 = prm;
    prm2(9) = y(10);                                   % 시변 버스 기준전압
    [uh, dgh] = prism_stageB_controller(y(1:9), prm2, init, tab, y(11), [double(y(14) == 1); y(15)]);
    if round(y(12)) == 3
        uh(1) = y(13);                                 % 전류 조향: 상태기계가 정한 변조율
    end
end
u = uh;
dg = dgh;
end

function [u, dg] = prism_stageB_controller(y, prm, init, tab, rst, aux)
%#codegen
%PRISM_STAGEB_CONTROLLER  Stage B 채택 제어기 1회 계산(제어주기 5 µs, 반송파 최댓값에서 표본).
%
%  검증 코드(model_stage_b_switching.run_core의 제어 부분)와 같은 법칙이다.
%   (1) 1주기 예측: 고속 상태 [i_p, v_s, i_h]를 직전 변조율로 5 µs 앞까지 공칭 모델로 적분(중점법 5단계)
%   (2) 상태궤환 + 버스전압 적분 → 브리지 전류지령(±84 A 포화, 역포화 보정)
%   (3) 내부 전류 법칙 → 변조율 m(±0.95)
%   (4) 링크전압 PI + 소비전류 앞먹임 → DAB 링크전류 지령(정격 80 A·8 kW·SPS 한계)
%   (5) DAB 링크전류 → 위상: 누설 인덕턴스 −10 % 기준 앞먹임 + 측정 전류비 ρ̂ 보정 + 저전류 가산 보정 ε̂
%   (6) H-브리지 데드타임 보상: 교정표 × 전류 스케줄 κ(20 A 이하 0.6 → 80 A 1.0)
%
%  입력
%   y    = [i_p v_s v_bus i_h v_link V_bat i_link_avg ph_c0 ph_c1]  (표본값)
%          i_link_avg : 직전 제어주기의 DAB 링크 직류전류 평균(측정)
%          ph_c0/ph_c1: 그 주기의 두 반주기 중심에서 적용된 유효 위상(게이트 생성기가 기록)
%   prm  = 상수 벡터(prism_hub_params의 P.ctrl_prm)
%           1 L  2 Cs  3 Cb  4 R  5 Lh  6 Rh  7 Clink  8 Ts  9 vref  10 vlink  11 mmax  12 refmax
%          13 link_max  14 power_max  15 link_bw  16 inner_tau  17 Ldab  18 fs  19 turns  20 phmax
%          21–25 K  26 lmin(0.9)  27 ρ̂ 이득  28 ρ̂ 최소 전류  29 ε̂ 이득  30 ε̂ 상한
%          31 κ 경부하 비율  32 κ 시작 전류  33 κ 1 도달 전류  34 교정표 기준 링크전압  35 예측 단계 수
%          36 예측 사용(1)  37 데드타임 보상 사용(1)
%   init = [q0 q_link0 m0 i_link0]   (평형점에서 시작: 적분기가 지령 = i_p가 되도록)
%   tab  = [i_grid; E(i)]            데드타임 교정표(전류별 상승 전이 한 번의 전압·시간 손실)
%   rst  = (선택, R2 창 조정 모듈 TB08) 1이면 이번 표본에서 무충격 재초기화한다. 적분기를 지령 = 경로전류가 되도록 맞추고
%          링크 적분기·직전 변조율·ρ̂·ε̂를 처음 값(0, 0, 1, 0)으로 둔다(검증 코드 StageBController.reset과 같은 계산).
%          영벡터·바이패스로 제어 출력이 쓰이지 않는 동안 매 표본 다시 맞춰, 제어를 시작할 때 충격이 없게 한다.
%          네 입력으로 부르면(TB04–TB07) 이 기능은 없고 계산은 이전과 같다.
%   aux  = (선택, R2 보호 상태기계 TB09) [보조 지령 사용(1/0); 보조 링크전류 지령 A]. 1이면 링크전압 PI 대신 보조 지령을
%          DAB 링크전류 지령으로 쓴다(H-브리지 차단 강등에서 상태기계의 보조 루프가 링크전압으로 버스를 붙잡을 때).
%          위상 계산(전류비·저전류 보정 포함)은 같다. 다섯 입력 이하로 부르면 이전과 같다.
%  출력
%   u  = [PWM 비교값(데드타임 보상 후); DAB 유효 위상 지령 rad]
%   dg = [m 지령(보상 전); 링크전류 지령; 브리지 전류지령; ρ̂; ε̂; 예측 링크전류]

persistent q qlink mprev rho epsA vbprev started
if isempty(started)
    q = init(1); qlink = init(2); mprev = init(3); rho = 1; epsA = 0; vbprev = y(3); started = 1;
end

L = prm(1); Cs = prm(2); R = prm(4); Lh = prm(5); Rh = prm(6); Clink = prm(7); Ts = prm(8);
vref = prm(9); vlink = prm(10); mmax = prm(11); refmax = prm(12);
link_max = prm(13); power_max = prm(14); link_bw = prm(15); itau = prm(16);
Ldab = prm(17); fs = prm(18); turns = prm(19); phmax = prm(20);
K = prm(21:25);
lmin = prm(26); est_g = prm(27); est_min = prm(28); eps_g = prm(29); eps_max = prm(30);
k_scale = prm(31); k_from = prm(32); k_full = prm(33); Vtab = prm(34); nsub = prm(35);

ip = y(1); vs = y(2); vb = y(3); ih = y(4); vl = y(5); vbat = y(6);
il_meas = y(7); ph_c0 = y(8); ph_c1 = y(9);
if nargin >= 5                                   % (R2, TB08) 무충격 재초기화
    if rst > 0.5
        q = -(ip + K(1)*ip + K(2)*vs + K(3)*vb + K(4)*ih)/K(5);
        qlink = 0; mprev = 0; rho = 1; epsA = 0; vbprev = vb;
    end
end

% ---- (1) 1주기 예측 -----------------------------------------------------------------
sip = ip; svs = vs; sih = ih;
if prm(36) > 0.5
    m = mprev; h = Ts/nsub;
    for s = 1:nsub
        a1 = (vbat/2 - R*sip + svs - vb)/L;
        a2 = (sih - sip)/Cs;
        a3 = (m*vl - svs - Rh*sih)/Lh;
        mp = sip + 0.5*h*a1;  mv = svs + 0.5*h*a2;  mh = sih + 0.5*h*a3;
        b1 = (vbat/2 - R*mp + mv - vb)/L;
        b2 = (mh - mp)/Cs;
        b3 = (m*vl - mv - Rh*mh)/Lh;
        sip = sip + h*b1;  svs = svs + h*b2;  sih = sih + h*b3;
    end
end
% ---- (2) 상태궤환 + 적분 -----------------------------------------------------------
raw  = -(K(1)*sip + K(2)*svs + K(3)*vb + K(4)*sih) - K(5)*q;
iref = min(refmax, max(-refmax, raw));
q = q + Ts*(vref - vb) + 0.1*(iref - raw)/(-K(5));
% ---- (3) 내부 전류 법칙 → 변조율 ---------------------------------------------------
vlx = max(vl, 1);                                % (보상 계산용 하한)
mraw = (svs + Rh*sih + Lh/itau*(iref - sih))/vl;
mcmd = min(mmax, max(-mmax, mraw));
% ---- (4) 링크전압 PI + 앞먹임 → DAB 링크전류 지령 ---------------------------------
w = 2*pi*link_bw;
rawlink = mcmd*sih + Clink*(2*0.7*w*(vlink - vl) + w*w*qlink);
sps = max(vb, 0)*turns*phmax*(1 - phmax/pi)/(2*pi*fs*Ldab);
lim = min(min(link_max, sps), power_max/max(vl, 1e-9));
icmd = min(lim, max(-lim, rawlink));
qlink = qlink + Ts*(vlink - vl) + 0.1*(icmd - rawlink)/(Clink*w*w);
if nargin >= 6                                   % (R2 보호, TB09) 보조 링크전류 지령
    if aux(1) > 0.5
        icmd = aux(2); qlink = 0;
    end
end
mprev = mcmd;
% ---- (5) DAB 전류비·저전류 보정 → 위상 ----------------------------------------------
% 직전 주기 두 반주기 중심에 적용된 위상의 예측 전류. 그 위상을 적용할 때 쓰인 버스전압은 직전 표본값이다
% (검증 모델: 반주기 중심에서 그때의 측정 버스전압으로 예측 전류를 계산).
il_pred = 0.5*(ipred(ph_c0, vbprev, turns, fs, Ldab, lmin) + ipred(ph_c1, vbprev, turns, fs, Ldab, lmin));
vbprev = vb;
dph = abs(ph_c1 - ph_c0);
if abs(il_pred) >= est_min && il_meas*il_pred > 0 && dph < 0.035
    rho = rho + est_g*(il_meas/il_pred - rho);
    rho = min(max(rho, 0.75), 1.25);
end
if eps_g > 0
    if abs(il_pred) < est_min && dph < 0.035
        epsA = epsA + eps_g*((il_meas - rho*il_pred) - epsA);
    elseif abs(il_pred) >= est_min
        epsA = epsA - eps_g*epsA;
    end
    epsA = min(max(epsA, -eps_max), eps_max);
end
ph_new = phase_ff((icmd - epsA)/rho, vb, turns, fs, Ldab, lmin, phmax);
% ---- (6) H-브리지 데드타임 보상 ----------------------------------------------------
m_pwm = mcmd;
if prm(37) > 0.5
    kap = k_scale + (1 - k_scale)*min(max((abs(sih) - k_from)/max(k_full - k_from, 1e-9), 0), 1);
    m_pwm = mcmd - kap*dt_error_tab(mcmd, sih, vlx, Lh, fs, tab, Vtab)/vlx;
end
u  = [m_pwm; ph_new];
dg = [mcmd; icmd; iref; rho; epsA; il_pred];
end

% ======================================================================================
function i = ipred(ph, vb, turns, fs, Ldab, lb)
% 위상 ph에서 SPS 식이 주는 링크전류(누설 인덕턴스 = 공칭의 lb배 가정)
k = turns*max(vb, 1)/(2*pi*fs*Ldab*lb);
i = k*ph*(1 - abs(ph)/pi);
end

function ph = phase_ff(il, vb, turns, fs, Ldab, lb, phmax)
% 링크전류 → SPS 위상 앞먹임(|φ| ≤ φ_max)
k = turns*max(vb, 1)/(2*pi*fs*Ldab*lb);
a = min(abs(il)/(pi*k/4), 1);
ph = min(pi/2*(1 - sqrt(1 - a)), phmax);
if il < 0, ph = -ph; end
end

function d = dt_error_tab(m, i, V, Lh, f, tab, Vtab)
% 유니폴라 PWM 한 주기의 브리지 평균 전압오차 [V]: 리플 극값 전류에서의 전이별 손실을 교정표에서 읽는다.
sg = 1;
if m < 0, m = -m; i = -i; sg = -1; end
r = V*m*(1 - m)/(4*Lh*f);
imin = i - r; imax = i + r;
d = sg*2*(tab_interp(-imax, tab) - tab_interp(imin, tab))*(V/Vtab)*f;
end

function e = tab_interp(x, tab)
% 선형 보간(범위 밖은 끝값) — numpy.interp와 같음
n = size(tab, 2);
if x <= tab(1, 1), e = tab(2, 1); return; end
if x >= tab(1, n), e = tab(2, n); return; end
lo = 1; hi = n;
while hi - lo > 1
    mid = floor((lo + hi)/2);
    if tab(1, mid) <= x, lo = mid; else, hi = mid; end
end
w = (x - tab(1, lo))/(tab(1, hi) - tab(1, lo));
e = tab(2, lo) + w*(tab(2, hi) - tab(2, lo));
end
